simulink model "turbo_controller"  (R2025a)
settings: Solver=FixedStepAuto  StartTime=0.0  StopTime=inf  FixedStep=0.001  RelTol=1e-3
PostLoadFcn:
  | % 自动定位同目录CubeMX文件；不需要外部初始化脚本。
  | codertarget.data.setParameterValue('turbo_controller','STM32CubeMX.ProjectFile',fullfile(fileparts(get_param('turbo_controller','FileName')),'turbo_f407.ioc'));
InitFcn:
  | % 中文说明：按原控制器字段与类型创建三组接口总线；控制参数已内嵌。
  | tc_names=["EValve_Cycle" "EValve_Open" "Eblast_Cycle" "Eblast_Open" "Motor_Cycle" "Motor_Open" "EValve_Enable" "Eblast_Enable" "Motor_Enable" "SWO_Firework" "SWO_BleedAir" "EngineState" "Flag_ECUReset_Clear" "Flag_ECUReset_Save" "Flag_Reset_Enable" "Accelerator" "Nc_dem" "Nc"]; tc_types=["uint16" "uint16" "uint16" "uint16" "uint16" "uint16" "uint8" "uint8" "uint8" "uint8" "uint8" "uint8" "uint8" "uint8" "uint8" "single" "single" "single"];
  | for tc_k=1:numel(tc_names)
  |  tc_e(tc_k)=Simulink.BusElement; tc_e(tc_k).Name=char(tc_names(tc_k)); tc_e(tc_k).DataType=char(tc_types(tc_k));
  | end
  | EngineControl_Out=Simulink.Bus; EngineControl_Out.DataScope='Exported'; EngineControl_Out.Elements=tc_e;
  | clear tc_e tc_names tc_types tc_k
  | tc_names=["savedata1" "savedata2" "savedata3" "savedata4" "savedata5" "savedata6" "savedata7" "savedata8" "savedata9" "savedata10" "savedata11" "savedata12" "savedata13" "savedata14" "savedata15" "savedata16" "savedata17" "savedata18" "savedata19" "savedata20" "savedata21" "savedata22" "savedata23" "savedata24" "savedata25"]; tc_types=["single" "single" "single" "single" "single" "single" "single" "single" "single" "single" "single" "single" "single" "single" "single" "single" "single" "single" "single" "single" "single" "single" "single" "single" "single"];
  | for tc_k=1:numel(tc_names)
  |  tc_e(tc_k)=Simulink.BusElement; tc_e(tc_k).Name=char(tc_names(tc_k)); tc_e(tc_k).DataType=char(tc_types(tc_k));
  | end
  | SaveData_Out=Simulink.Bus; SaveData_Out.DataScope='Exported'; SaveData_Out.Elements=tc_e;
  | clear tc_e tc_names tc_types tc_k
  | tc_names=["senddata1" "senddata2" "senddata3" "senddata4" "senddata5" "senddata6" "senddata7" "senddata8" "senddata9" "senddata10" "senddata11" "senddata12" "senddata13" "senddata14" "senddata15" "senddata16" "senddata17" "senddata18" "senddata19" "senddata20" "senddata21" "senddata22" "senddata23" "senddata24" "senddata25" "senddata26" "senddata27" "senddata28" "senddata29"]; tc_types=["uint8" "uint8" "uint8" "uint8" "uint8" "uint8" "uint8" "uint8" "uint8" "uint8" "uint8" "uint8" "uint8" "uint8" "uint8" "uint8" "uint8" "uint8" "uint8" "uint8" "uint8" "uint8" "uint8" "uint8" "uint8" "uint8" "uint8" "uint8" "uint8"];
  | for tc_k=1:numel(tc_names)
  |  tc_e(tc_k)=Simulink.BusElement; tc_e(tc_k).Name=char(tc_names(tc_k)); tc_e(tc_k).DataType=char(tc_types(tc_k));
  | end
  | SendData_Out=Simulink.Bus; SendData_Out.DataScope='Exported'; SendData_Out.Elements=tc_e;
  | clear tc_e tc_names tc_types tc_k
  | 
  | % 以下为接口中文说明；只设置描述，不改变数值或数据类型。
  | EngineControl_Out.Description='执行控制输出（阀、电机、点火、状态及复位请求）';
  | tc_cn=["EValve_Cycle（主油阀周期计数（每计数2毫秒））" "EValve_Open（主油阀开通计数（每计数2毫秒））" "Eblast_Cycle（副油阀周期计数（每计数2毫秒））" "Eblast_Open（副油阀开通计数（每计数2毫秒））" "Motor_Cycle（起动电机周期计数）" "Motor_Open（起动电机开通计数）" "EValve_Enable（主油阀驱动使能）" "Eblast_Enable（副油阀驱动使能）" "Motor_Enable（起动电机使能）" "SWO_Firework（点火器使能（1开））" "SWO_BleedAir（引气阀使能（1开））" "EngineState（发动机状态）" "Flag_ECUReset_Clear（清除复位恢复状态请求）" "Flag_ECUReset_Save（保存复位恢复数据请求）" "Flag_Reset_Enable（处理器软件复位请求）" "Accelerator（油门／油泵给定控制量）" "Nc_dem（控制目标转速）" "Nc（发动机反馈转速（转每分））"];
  | tc_elements=EngineControl_Out.Elements;
  | for tc_k=1:numel(tc_cn)
  |  tc_elements(tc_k).Description=char(tc_cn(tc_k));
  | end
  | EngineControl_Out.Elements=tc_elements;
  | clear tc_cn tc_elements tc_k
  | SaveData_Out.Description='25项运行记录；字段含义按当前模型数据来源解释';
  | tc_cn=["savedata1（指令回显记录）" "savedata2（入口总温记录（℃））" "savedata3（电源电压记录）" "savedata4（排气温度记录（℃））" "savedata5（标定燃油压力记录）" "savedata6（副油阀占空比记录（％））" "savedata7（主油阀占空比记录（％））" "savedata8（温度修正转速记录）" "savedata9（开关输出及反馈位域）" "savedata10（物理转速记录）" "savedata11（油泵目标给定原始值）" "savedata12（起动电机占空比记录（％））" "savedata13（发动机状态码记录）" "savedata14（故障告警位域记录）" "savedata15（模型记录帧序号）" "savedata16（处理器温度记录（℃））" "savedata17（装订转速记录（沿用旧电源字段名））" "savedata18（导航高度记录）" "savedata19（飞行空速记录）" "savedata20（主阀旧记录位（恒零保留））" "savedata21（第21项保留记录（恒零））" "savedata22（保留记录项22）" "savedata23（保留记录项23）" "savedata24（保留记录项24）" "savedata25（保留记录项25）"];
  | tc_elements=SaveData_Out.Elements;
  | for tc_k=1:numel(tc_cn)
  |  tc_elements(tc_k).Description=char(tc_cn(tc_k));
  | end
  | SaveData_Out.Elements=tc_elements;
  | clear tc_cn tc_elements tc_k
  | SendData_Out.Description='29字段回传及外设命令接口；板端上位机帧只取第3至27字段';
  | tc_cn=["senddata1（回传发送允许标志（不直接上线路））" "senddata2（回传载荷长度25字节）" "senddata3（回传指令回显字节）" "senddata4（总温编码字节（℃＋80））" "senddata5（电源电压编码字节）" "senddata6（排温编码高字节）" "senddata7（排温编码低字节）" "senddata8（燃油压力编码高字节）" "senddata9（燃油压力编码低字节）" "senddata10（副油阀占空比字节（％））" "senddata11（主油阀占空比字节（％））" "senddata12（修正转速编码高字节）" "senddata13（修正转速编码低字节）" "senddata14（驱动及反馈状态位域）" "senddata15（物理转速编码高字节）" "senddata16（物理转速编码低字节）" "senddata17（油泵目标给定高字节（串口二使用））" "senddata18（油泵目标给定低字节（串口二使用））" "senddata19（起动电机占空比命令（串口一使用））" "senddata20（发动机状态码字节）" "senddata21（故障告警位域字节）" "senddata22（帧序号占位（板端另行填写））" "senddata23（处理器温度编码（℃＋50））" "senddata24（控制目标转速编码高字节）" "senddata25（控制目标转速编码低字节）" "senddata26（占位字节（板端改填实测泵速高字节））" "senddata27（占位字节（板端改填实测泵速低字节））" "senddata28（装订转速高字节（本板未发送））" "senddata29（装订转速低字节（本板未发送））"];
  | tc_elements=SendData_Out.Elements;
  | for tc_k=1:numel(tc_cn)
  |  tc_elements(tc_k).Description=char(tc_cn(tc_k));
  | end
  | SendData_Out.Elements=tc_elements;
  | clear tc_cn tc_elements tc_k
  | 
  | 
  | % FRAM模块化事务：接口类型和上电初始状态，随模型保存，无外部初始化文件。
  | clear FM_elements
  | FM_elements(1)=Simulink.BusElement;FM_elements(1).Name='phase';FM_elements(1).DataType='uint8';FM_elements(1).Dimensions=[1 1];FM_elements(1).Description='phase（当前事务阶段）';
  | FM_elements(2)=Simulink.BusElement;FM_elements(2).Name='a';FM_elements(2).DataType='uint8';FM_elements(2).Dimensions=[64 1];FM_elements(2).Description='a（启动时缓存的首区64字节）';
  | FM_elements(3)=Simulink.BusElement;FM_elements(3).Name='active';FM_elements(3).DataType='uint16';FM_elements(3).Dimensions=[1 1];FM_elements(3).Description='active（当前有效记录区地址）';
  | FM_elements(4)=Simulink.BusElement;FM_elements(4).Name='generation';FM_elements(4).DataType='uint32';FM_elements(4).Dimensions=[1 1];FM_elements(4).Description='generation（当前有效记录代号）';
  | FM_elements(5)=Simulink.BusElement;FM_elements(5).Name='record';FM_elements(5).DataType='uint8';FM_elements(5).Dimensions=[64 1];FM_elements(5).Description='record（本次冻结的待写记录）';
  | FM_elements(6)=Simulink.BusElement;FM_elements(6).Name='addr';FM_elements(6).DataType='uint16';FM_elements(6).Dimensions=[1 1];FM_elements(6).Description='addr（本次备用写入地址）';
  | FM_elements(7)=Simulink.BusElement;FM_elements(7).Name='lastSave';FM_elements(7).DataType='single';FM_elements(7).Dimensions=[1 1];FM_elements(7).Description='lastSave（上次开始保存的秒数）';
  | FM_elements(8)=Simulink.BusElement;FM_elements(8).Name='lastState';FM_elements(8).DataType='uint8';FM_elements(8).Dimensions=[1 1];FM_elements(8).Description='lastState（上次保存时的发动机状态）';
  | FM_elements(9)=Simulink.BusElement;FM_elements(9).Name='boot';FM_elements(9).DataType='boolean';FM_elements(9).Dimensions=[1 1];FM_elements(9).Description='boot（启动记录是否允许恢复）';
  | FM_elements(10)=Simulink.BusElement;FM_elements(10).Name='consumed';FM_elements(10).DataType='boolean';FM_elements(10).Dimensions=[1 1];FM_elements(10).Description='consumed（本次启动恢复通知是否已发送）';
  | FM_elements(11)=Simulink.BusElement;FM_elements(11).Name='payload';FM_elements(11).DataType='uint8';FM_elements(11).Dimensions=[20 1];FM_elements(11).Description='payload（当前20字节恢复内容）';
  | ... (+35 lines)
model workspace (MAT data in the model file):
  CRC16_Table_Reference = [0 4129 8258 12387 16516 20645 24774 28903 33032 37161 41290 45419 ... (256 elements, 256x1)]
  PE_Kaer = [0.15402 0.15402 0.12264 0.10076 0.09481 0.07601 0.07111 0.0569 0.05198 0.04926 0.05308 0.04325 ... (13 elements, 1x13)]
  PE_Nr = [21.2982 61.4260372 67.7475458 72.7394382 76.845934 80.6988798 83.8449282 86.6491912 88.9382406 89.178606 91.1938214 93.4068058 ... (13 elements, 1x13)]
  PE_Pump_Translate = 33.5999984741
  PE_RotaSpeed_Translate = 860
  PE_Taer = [0.4939154 0.4939154 0.40780982 0.34066978 0.31622756 0.30405716 0.34300244 0.26785022 0.37393554 0.23914836 0.44563948 0.31044662 ... (13 elements, 1x13)]
  PF_ACCFULLRANGE = 3360
  PF_Flag_ECUReset = 0
  PF_Flag_rx_suc = 1
  PF_Gear_Info = [40000; 45000; 50000; 55000; 57000; 59000; 60000; 61000; 61000; 61000; 61000; 61000]
  PF_K_TiaoJie = 1
  PF_Kpu = 10
  PF_MySet_Rxdata = [0 0 0 0 0 0 0 0 0 0 0 0 ... (50 elements, 50x1)]
  PF_MyUsart1_Rxdata = [0 0 0 0 0 0 0 0 0 0 0 0 ... (50 elements, 50x1)]
  PF_MyUsart2_Rxdata = [0 0 0 0 0 0 0 0 0 0 0 0 ... (50 elements, 50x1)]
  PF_Reset_Information = [0 0 0 0 0 0 0 0 0 0 0 0 ... (20 elements, 20x1)]
  PF_Sensor_X1_T4 = [0 4095]
  PF_Sensor_X2_T4 = [0 1.66666698456]
  PF_Sensor_X3_T4 = [0 504 999 1497 2010 2529 3051 3568 4076 4571 4959]
  PF_Sensor_X_P2 = [0.5 3]
  PF_Sensor_X_Poil = [0.5 3]
  PF_Sensor_X_T1t = [-50 300]
  PF_Sensor_X_Vpower = [0 3]
  PF_Sensor_X_Vpump = [0 3]
  PF_Sensor_Y1_T4 = [0 3]
  PF_Sensor_Y2_T4 = [0 5000]
  PF_Sensor_Y3_T4 = [0 100 200 300 400 500 600 700 800 900 980]
  PF_Sensor_Y_P2 = [0 1000]
  PF_Sensor_Y_Poil = [0 1000]
  PF_Sensor_Y_T1t = [-50 300]
  PF_Sensor_Y_Vpower = [0 33]
  PF_Sensor_Y_Vpump = [0 33]
  PG_CtrlMode_CloseLoop : mpt.Parameter (value not decoded)
  PG_CtrlMode_ManualAcc : mpt.Parameter (value not decoded)
  PG_CtrlMode_Origin : mpt.Parameter (value not decoded)
  PG_CtrlMode_Start : mpt.Parameter (value not decoded)
  PG_CtrlMode_Stop : mpt.Parameter (value not decoded)
  PG_ES_Clp : mpt.Parameter (value not decoded)
  PG_ES_EngStart : mpt.Parameter (value not decoded)
  PG_ES_Manual : mpt.Parameter (value not decoded)
  PG_ES_Origin : mpt.Parameter (value not decoded)
  PG_ES_Stop : mpt.Parameter (value not decoded)
  PG_Instr_BleedAirSet : mpt.Parameter (value not decoded)
  PG_Instr_CloseLoop : mpt.Parameter (value not decoded)
  PG_Instr_ECUReSet : mpt.Parameter (value not decoded)
  PG_Instr_EValveSet : mpt.Parameter (value not decoded)
  PG_Instr_EblastSet : mpt.Parameter (value not decoded)
  PG_Instr_Erase : mpt.Parameter (value not decoded)
  PG_Instr_FireWorkSet : mpt.Parameter (value not decoded)
  PG_Instr_ManualPlus : mpt.Parameter (value not decoded)
  PG_Instr_ManualrReduce : mpt.Parameter (value not decoded)
  PG_Instr_MotorSet : mpt.Parameter (value not decoded)
  PG_Instr_OilSet : mpt.Parameter (value not decoded)
  PG_Instr_SelfCheck : mpt.Parameter (value not decoded)
  PG_Instr_Start : mpt.Parameter (value not decoded)
  PG_Instr_Stop : mpt.Parameter (value not decoded)
  PG_Instr_StopZero : Simulink.Parameter (value not decoded)
  PG_Location_Air : Simulink.Parameter (value not decoded)
  PG_Location_Gnd : Simulink.Parameter (value not decoded)
  PG_ServoCtrlMode_CloseLoop : Simulink.Parameter (value not decoded)
  PG_ServoCtrlMode_CloseLoopMax : Simulink.Parameter (value not decoded)
  PG_ServoCtrlMode_CloseLoopMin : Simulink.Parameter (value not decoded)
  PG_ServoCtrlMode_ManualAcc : Simulink.Parameter (value not decoded)
  PG_ServoCtrlMode_ManualAccMax : Simulink.Parameter (value not decoded)
  PG_ServoCtrlMode_ManualAccMin : Simulink.Parameter (value not decoded)
  PG_SpeedDot_Permit : Simulink.Parameter (value not decoded)
  PL_EngineModel_Actuator = [0 10 100]
  PL_EngineModel_EngineStar_Press_P2 = [1013 1098.4 1099.144828 1099.931034 1103.613793 1162.662069 1143.793103 1131.006897 1123.186207 1117.6 1114 1111.806897 ... (127 elements, 1x127)]
  PL_EngineModel_EngineStar_RotaSpeed = [200 2000 9584 9660 10220 10240 10260 10288 10308 10368 10380 10408 ... (127 elements, 1x127)]
  PL_EngineModel_EngineStar_Temp_Exhaust = [128 129 129.1 130 131 131.1 132 133 134 134.1 135 135.1 ... (127 elements, 1x127)]
  PL_EngineModel_EngineStar_Time = [0.05 0.1 0.15 0.2 0.25 0.3 0.35 0.4 0.45 0.5 0.55 0.6 ... (127 elements, 1x127)]
  PL_EngineModel_IdleAbove_Nr = [0 21.2982 61.4260372 67.7475458 72.7394382 76.845934 80.6988798 83.8449282 86.6491912 88.9382406 89.178606 91.1938214 ... (14 elements, 1x14)]
  PL_EngineModel_IdleAbove_P2r = [0.986923266716 1.57907722675 1.81593881076 1.99358499877 2.23044658278 2.43770046879 2.65482358747 2.84233900814 3.03972366149 3.18776215149 3.25684678016 3.3950160375 ... (14 elements, 1x14)]
  PL_EngineModel_IdleAbove_Tempr = [0.0536001429337 1.07200285867 1.63301768805 1.63659103091 1.66875111667 1.72592460247 1.77595140254 1.86171163123 1.95461854565 2.03323208862 2.03323208862 2.13685903162 ... (14 elements, 1x14)]
  PL_EngineModel_IdleAbove_Ter = [0.42434128 0.42434128 0.42434128 0.30669408 0.23570008 0.22150128 0.1997974 0.23803274 0.16115638 0.24279948 0.13600422 0.31308354 ... (14 elements, 1x14)]
  PL_EngineModel_IdleAbove_Wfr = [0 10.142 23.8337 27.8905 31.9473 36.0041 40.0609 44.1177 48.1745 52.2313 52.7384 56.7952 ... (14 elements, 1x14)]
  PL_EngineModel_Press_P2 = [400 400 400 400 400 400 400 400 400 400]
  PL_EngineModel_Rotaspeed = [0 20000 96400]
  PL_EngineModel_Temp_Exhaust = [500 500 500 500 500 500 500 500 500 500]
  PL_Kaer = [0.1 0.1 0.1 0.1 0.1 0.1]
  PL_Nr = [50 60 70 80 90 100]
  PL_Taer = [0.1 0.1 0.1 0.1 0.1 0.1]
  Sig : Simulink.Signal (value not decoded)
  Ts_ms : Simulink.Parameter (value not decoded)
  false : Simulink.Parameter (value not decoded)
  true : Simulink.Parameter (value not decoded)
symbols that are objects in the model workspace (value not decoded): PG_CtrlMode_CloseLoop, PG_CtrlMode_ManualAcc, PG_CtrlMode_Origin, PG_CtrlMode_Start, PG_CtrlMode_Stop, PG_ES_Clp, PG_ES_EngStart, PG_ES_Manual, PG_ES_Origin, PG_ES_Stop, PG_Instr_BleedAirSet, PG_Instr_CloseLoop, PG_Instr_EblastSet, PG_Instr_ECUReSet, PG_Instr_Erase, PG_Instr_EValveSet, PG_Instr_FireWorkSet, PG_Instr_ManualPlus, PG_Instr_ManualrReduce, PG_Instr_MotorSet, PG_Instr_OilSet, PG_Instr_SelfCheck, PG_Instr_Start, PG_Instr_Stop, PG_Instr_StopZero, PG_ServoCtrlMode_CloseLoop, PG_ServoCtrlMode_CloseLoopMax, PG_ServoCtrlMode_CloseLoopMin, PG_ServoCtrlMode_ManualAcc, PG_ServoCtrlMode_ManualAccMax, PG_ServoCtrlMode_ManualAccMin, Ts_ms
libraries: simulink x97, stm32blockslib x10, stm32f4xxblockslib x8
(part 16 of 26)

== system turbo_controller/COMMRead_ISM/ECUReset_Information_Read/ECUReset_Acclerator_Cal ==
  note: 把保存的两个字节还原成油泵给定
      |
      | 按高字节在前合成：泵给定=高字节×256+低字节。例如高字节11、低字节184，恢复得到3000。
      |
      | 这里只恢复无符号控制编码，不换算成燃油流量，不根据电压补偿，也不验证整条FRAM记录。记录校验
      | 、恢复是否允许和最终是否采用该值在事务层及父级完成。输入字段位置按恢复信息协议排列，不能随
      | 意调换高低字节。
  S_ECUReset_Information : Inport
      settings: AttributesFormatString=S_ECUReset_Information（铁电存储器中的复位恢复记录）
  ECUReset_Information_Acclerator1 : Selector  IndexMode=Zero-based  InputPortWidth=20  IndexOptions=Index vector (dialog)  Indices=[6]  OutputSizes=1
      settings: AttributesFormatString=ECUReset_Information_Acclerator1（控制器复位信息油门1）
  ECUReset_Information_Acclerator2 : Selector  IndexMode=Zero-based  InputPortWidth=20  IndexOptions=Index vector (dialog)  Indices=[7]  OutputSizes=1
      settings: AttributesFormatString=ECUReset_Information_Acclerator2（控制器复位信息油门2）
  Product20 : Product  Inputs=**
      settings: AttributesFormatString=Product20（乘法20）
  Sum of Elements3 : Sum
      settings: AttributesFormatString=Sum of Elements3（加法求和的元素3）
  dth = T0-288.24 : Constant  Value=256  OutDataTypeStr=single  SampleTime=-1
      settings: AttributesFormatString=dth = T0-288.24（固定常量256（旧名称不参与计算））
  S_ECUReset_Acclerator : Outport
      settings: AttributesFormatString=S_ECUReset_Acclerator（电子控制器复位油门）
  wires:
  Sum of Elements3/1 -> S_ECUReset_Acclerator/1
  ECUReset_Information_Acclerator1/1 -> Product20/1
  dth = T0-288.24/1 -> Product20/2
  Product20/1 -> Sum of Elements3/1
  ECUReset_Information_Acclerator2/1 -> Sum of Elements3/2
  S_ECUReset_Information/1 -> ECUReset_Information_Acclerator2/1, ECUReset_Information_Acclerator1/1

== system turbo_controller/COMMRead_ISM/ECUReset_Information_Read/Flag_ECUReset_Manage ==
  note: 还原保存的目标转速，并判定可否采用
      |
      | 从恢复信息中取出三个字节，高字节在前合成：
      | 目标rpm=高字节×65536+中字节×256+低字节。
      | 例如0、195、80合成50000。
      |
      | 目标在30000～89000之间才满足本模块的数值范围要求，再与外部恢复有效标志组合，形成恢复使用许
      | 可。范围合法仅说明数值像一个允许的目标，不能代替FRAM记录校验；外部标志为假时仍不采用。
      |
      | 目标输出继续送SpeedLoad_Analyse，最终还取决于当前模式和恢复选择。当前上层使能固定false，因
      | 此本模块的解码结果不会自行激活闭环。
  S_ECUReset_Information : Inport
      settings: AttributesFormatString=S_ECUReset_Information（铁电存储器中的复位恢复记录）
  S_Flag_ECUReset : Inport  Port=2
      settings: AttributesFormatString=S_Flag_ECUReset（复位恢复标志）
  ECUReset_Information_NcDem1 : Selector  IndexMode=Zero-based  InputPortWidth=20  IndexOptions=Index vector (dialog)  Indices=[10]  OutputSizes=1
      settings: AttributesFormatString=ECUReset_Information_NcDem1（控制器复位信息目标转速1）
  ECUReset_Information__NcDem2 : Selector  IndexMode=Zero-based  InputPortWidth=20  IndexOptions=Index vector (dialog)  Indices=[11]  OutputSizes=1
      settings: AttributesFormatString=ECUReset_Information__NcDem2（控制器复位信息目标转速2）
  ECUReset_Information__NcDem3 : Selector  IndexMode=Zero-based  InputPortWidth=20  IndexOptions=Index vector (dialog)  Indices=[12]  OutputSizes=1
      settings: AttributesFormatString=ECUReset_Information__NcDem3（控制器复位信息目标转速3）
  Logical Operator2 : Logic  AllPortsSameDT=off  OutDataTypeStr=boolean
      settings: AttributesFormatString=Logical Operator2（逻辑运算2）
  Logical Operator_ReSet : Logic  AllPortsSameDT=off  OutDataTypeStr=boolean
      settings: AttributesFormatString=Logical Operator_ReSet（逻辑运算复位）
  Product1 : Product  Inputs=**
      settings: AttributesFormatString=Product1（乘法1）
  Product2 : Product  Inputs=**
      settings: AttributesFormatString=Product2（乘法2）
  Relational Operator1 : RelationalOperator  OutDataTypeStr=boolean  InputSameDT=off
      settings: AttributesFormatString=Relational Operator1（关系比较运算1）
  Relational Operator6 : RelationalOperator  Operator=<=  OutDataTypeStr=boolean  InputSameDT=off
      settings: AttributesFormatString=Relational Operator6（关系比较运算6）
  Sum of Elements1 : Sum  Inputs=+++
      settings: AttributesFormatString=Sum of Elements1（加法求和的元素1）
  ZhuangDingShangXian_uint32 : Constant  Value=89000  OutDataTypeStr=uint32
      settings: AttributesFormatString=ZhuangDingShangXian_uint32（装订上限三十二位无符号整数）
  ZhuangDingXiaXian_uint32 : Constant  Value=30000  OutDataTypeStr=uint32
      settings: AttributesFormatString=ZhuangDingXiaXian_uint32（装订下限三十二位无符号整数）
  dth = T0-288.1 : Constant  Value=256  OutDataTypeStr=single  SampleTime=-1
      settings: AttributesFormatString=dth = T0-288.1（固定常量256（旧名称不参与计算））
  dth = T0-288.2 : Constant  Value=65536  OutDataTypeStr=single  SampleTime=-1
      settings: AttributesFormatString=dth = T0-288.2（固定常量65536（旧名称不参与计算））
  S_Flag_ECUReset_Process : Outport
      settings: AttributesFormatString=S_Flag_ECUReset_Process（标志控制器复位处理）
  S_ECUReset_NcDem : Outport  Port=2
      settings: AttributesFormatString=S_ECUReset_NcDem（电子控制器复位目标转速）
  wires:
  Logical Operator2/1 -> S_Flag_ECUReset_Process/1
  S_ECUReset_Information/1 -> ECUReset_Information_NcDem1/1, ECUReset_Information__NcDem3/1, ECUReset_Information__NcDem2/1
  Relational Operator6/1 -> Logical Operator_ReSet/2
  Relational Operator1/1 -> Logical Operator_ReSet/1
  ZhuangDingShangXian_uint32/1 -> Relational Operator6/2
  ZhuangDingXiaXian_uint32/1 -> Relational Operator1/2
  dth = T0-288.1/1 -> Product1/2
  ECUReset_Information__NcDem2/1 -> Product1/1
  ECUReset_Information__NcDem3/1 -> Sum of Elements1/3
  Product1/1 -> Sum of Elements1/2
  Product2/1 -> Sum of Elements1/1
  ECUReset_Information_NcDem1/1 -> Product2/1
  dth = T0-288.2/1 -> Product2/2
  Sum of Elements1/1 -> S_ECUReset_NcDem/1, Relational Operator6/1, Relational Operator1/1
  Logical Operator_ReSet/1 -> Logical Operator2/1
  S_Flag_ECUReset/1 -> Logical Operator2/2

== system turbo_controller/COMMRead_ISM/ISM/AnalogFilter_Nc ==
  note: 检查转速可信度，并形成控制转速及相对转速
      |
      | 先按模式设置转速下限：闭环时采用10000，其他模式采用0；上限70000。GeneralFilter同时检查相邻
      | 两拍变化，突变量门限1200、恢复门限800、恢复确认参数100 ms。
      |
      | 异常样本可能被上一有效值替代，然后进行一阶低通，得到Nc_Filter。范围故障与变化故障分别输出
      | ，供FPM决定暂时保持控制还是采用故障备份曲线。
      |
      | 相对转速以61000 rpm为100%：百分比=当前转速×100/61000。另有按温度sqrt(288.15/T1t_calc)修正
      | 的转速及百分比。温度必须为K；当前此输入由上层接288.15 K，修正系数为1。不要与独立的ADC总温
      | 修正记录通道混淆。
  T1t_calc : Inport
      settings: AttributesFormatString=T1t_calc（入口总温计算）
  S_Nc : Inport  Port=2
      settings: AttributesFormatString=S_Nc（发动机反馈转速（转每分））
  S_EngineState : Inport  Port=3
      settings: AttributesFormatString=S_EngineState（发动机状态）
  Constant1 : Constant  Value=0  OutDataTypeStr=single  SampleTime=-1
      settings: AttributesFormatString=Constant1（常量1）
  Constant2 : Constant  Value=70000  OutDataTypeStr=single  SampleTime=-1
      settings: AttributesFormatString=Constant2（常量2）
  Constant3 : Constant  Value=10000  OutDataTypeStr=single  SampleTime=-1
      settings: AttributesFormatString=Constant3（常量3）
  Constant4 : Constant  Value=1200  OutDataTypeStr=single  SampleTime=-1
      settings: AttributesFormatString=Constant4（常量4）
  Constant5 : Constant  Value=800  OutDataTypeStr=single  SampleTime=-1
      settings: AttributesFormatString=Constant5（常量5）
  Constant6 : Constant  Value=100  OutDataTypeStr=single  SampleTime=-1
      settings: AttributesFormatString=Constant6（常量6）
  GeneralFilter : Subsystem  Description=|  RequirementInfo={} %GIDa_36ea9eb8_e302_4863_9c8a_4518a6f49dc1
      | 先拒绝明显不可信的转速，再平滑有效值
      | 
      | Xlim_Xdot_Judge比较当前原始输入、前一拍原始输入和前一拍有效输出。超出允许上下限或突变不满足接受条件时，输出沿用上次有效值，并分别标记幅值故障、变化故障。
      | 
      | 恢复时不仅要求变化回到较小门限，还要达到连续确认次数。次数由恢复时间/Ts_ms计算，避免一拍恢复就马上解除故障。
      | 
      | 通过检查的值再进入一阶低通，延迟同时保存本拍原始值和有效值，供下一拍比较。因此“原始上一拍”与“上一有效输出”是两条不同的记忆，不能混为一个变量。
      settings: AttributesFormatString=GeneralFilter（通用滤波）
  N1r_idle1 : Constant  Value=PG_ES_Clp  OutDataTypeStr=uint8  SampleTime=-1
      settings: AttributesFormatString=N1r_idle1（一级转速归一化值慢车1）
  Product1 : Product  Inputs=**/
      settings: AttributesFormatString=Product1（乘法1）
  Product2 : Product  Inputs=*/
      settings: AttributesFormatString=Product2（乘法2）
  Product3 : Product  Inputs=**
      settings: AttributesFormatString=Product3（乘法3）
  Product4 : Product  Inputs=**
      settings: AttributesFormatString=Product4（乘法4）
  Relational Operator4 : RelationalOperator  Operator===  OutDataTypeStr=boolean  InputSameDT=off
      settings: AttributesFormatString=Relational Operator4（关系比较运算4）
  Sqrt : Sqrt
      settings: AttributesFormatString=Sqrt（平方根）
  Switch : Switch  Criteria=u2 ~= 0  SaturateOnIntegerOverflow=off  InputSameDT=off
      settings: AttributesFormatString=Switch（开关选择）
  constant1 : Constant  Value=single(288.15)  OutDataTypeStr=single  SampleTime=-1
      settings: AttributesFormatString=constant1（常量1）
  constant2 : Constant  Value=100  OutDataTypeStr=single  SampleTime=-1
      settings: AttributesFormatString=constant2（常量2）
  constant3 : Constant  Value=61000  OutDataTypeStr=single  SampleTime=-1
      settings: AttributesFormatString=constant3（常量3）
  Nc_Flag_Locking : Outport
      settings: AttributesFormatString=Nc_Flag_Locking（转速标志锁存）
  Ncdot_Flag_Locking : Outport  Port=2
      settings: AttributesFormatString=Ncdot_Flag_Locking（控制器转速变化量标志锁存）
  Nc_Filter : Outport  Port=3
      settings: AttributesFormatString=Nc_Filter（滤波后的转速）
  Nc_Percent : Outport  Port=4
      settings: AttributesFormatString=Nc_Percent（转速百分比）
  Ncr : Outport  Port=5
      settings: AttributesFormatString=Ncr（归一化控制器转速）
  Ncr_Percent : Outport  Port=6
      settings: AttributesFormatString=Ncr_Percent（归一化控制器转速百分比）
  wires:
  GeneralFilter/3(S_Xout) -> Product3/1, Product1/1, Nc_Filter/1  "Nc（反馈转速）"
  Constant4/1 -> GeneralFilter/4(Xdot_lim)
  GeneralFilter/1(S_X_Flag_Locking) -> Nc_Flag_Locking/1  "X_Flag_Locking（输入信号锁定标志）"
  Constant2/1 -> GeneralFilter/2(X_ulim)
  S_Nc/1 -> GeneralFilter/1(Xin)
  Constant6/1 -> GeneralFilter/6(Xdot_CancelTime)
  GeneralFilter/2(S_Xdot_Flag_Locking) -> Ncdot_Flag_Locking/1  "Xdot_Flag_Locking（输入变化率锁定标志）"
  Switch/1 -> GeneralFilter/3(X_llim)
  Constant5/1 -> GeneralFilter/5(Xdot_CancelLim)
  Product1/1 -> Product4/1, Nc_Percent/1  "Nc_Percent（转速百分比）"
  constant2/1 -> Product1/2
  constant3/1 -> Product1/3
  constant1/1 -> Product2/1
  T1t_calc/1 -> Product2/2
  Product2/1 -> Sqrt/1
  Sqrt/1 -> Product3/2, Product4/2
  Product4/1 -> Ncr_Percent/1  "Ncr_Percent（归一化控制器转速百分比）"
  Product3/1 -> Ncr/1  "Ncr（归一化控制器转速）"
  N1r_idle1/1 -> Relational Operator4/2
  S_EngineState/1 -> Relational Operator4/1
  Constant1/1 -> Switch/3
  Constant3/1 -> Switch/1
  Relational Operator4/1 -> Switch/2

== system turbo_controller/COMMRead_ISM/ISM/AnalogFilter_Poil ==
  note: 对标定后的油压做一阶低通，减小采样抖动
      |
      | 每次把本拍输入与上次滤波结果按比例相加：
      | 本拍输出=α×本拍输入+β×上次输出；
      | α=Ts/(T+Ts)，β=T/(T+Ts)。
      |
      | 当前T=0.067 s，Ts=Ts_ms/1000=0.02 s，因此α约0.229885、β约0.770115。新输入约占23%，旧结果
      | 约占77%。例如上次输出100、本次输入200，本次滤波结果约123，随后逐步靠近200。
      |
      | 它抑制快速波动，也会让真实变化稍有滞后；不负责把ADC计数变成物理量，也不单凭滤波判定传感器
      | 故障。输出送POil_Filter，供起动阶段比较压力建立情况并用于记录。
  In1 : Inport
      settings: AttributesFormatString=In1（输入1）
  Constant7 : Constant  Value=Ts_ms  OutDataTypeStr=single  SampleTime=-1
      settings: AttributesFormatString=Constant7（常量7）
  Constant8 : Constant  Value=1000  OutDataTypeStr=single  SampleTime=-1
      settings: AttributesFormatString=Constant8（常量8）
  Constant9 : Constant  Value=single(0.067)  OutDataTypeStr=single  SampleTime=-1
      settings: AttributesFormatString=Constant9（常量9）
  Divide : Product  Inputs=*/
      settings: AttributesFormatString=Divide（除法）
  Integer Delay1 : Delay  DelayLength=1  InitialCondition=0
      settings: AttributesFormatString=Integer Delay1（整数延迟1）
  Product2 : Product  RndMeth=Zero
      settings: AttributesFormatString=Product2（乘法2）
  Product3 : Product  RndMeth=Zero
      settings: AttributesFormatString=Product3（乘法3）
  Subsystem1 : Subsystem  Description=|
      | 计算低通滤波中新样本的权重
      | 
      | 输入T为滤波时间常数（s），T_Sampling为采样周期（s）。输出α=T_Sampling/(T+T_Sampling)，供父级乘以本拍的新输入。
      | 
      | 当前T=0.067、采样周期0.02，α=0.02/0.087≈0.229885。也就是每拍只采用约23%的新值，另外约77%由历史结果补足。时间常数越大，新值权重越小，结果越平稳但响应越慢。
      | 
      | 本模块只算一个无量纲系数，不含延迟，也不直接输出温度、压力或转速。两项时间输入必须使用同一单位。
      settings: AttributesFormatString=Subsystem1（子系统1）
      mask Display: disp('T_S\n---------------\nT_S + T')
  Subsystem2 : Subsystem  Description=|
      | 计算低通滤波中历史结果的权重
      | 
      | 输入T为时间常数，T_Sampling为采样周期，两者都用s。输出β=T/(T+T_Sampling)，供父级乘以上一次滤波结果。
      | 
      | 当前T=0.067、采样周期0.02，β≈0.770115；与另一支路新样本权重α≈0.229885相加为1。这样常值输入最终会稳定在原值，不会因为反复相加而不断放大。
      | 
      | 本模块只计算系数，历史结果由父级延迟块保存。若把20 ms误传成20 s，权重和滤波速度都会完全改变，因此父级先将Ts_ms除以1000。
      settings: AttributesFormatString=Subsystem2（子系统2）
      mask Display: disp('T\n---------------\nT_S + T')
  Sum3 : Sum  Inputs=|++
      settings: AttributesFormatString=Sum3（加法求和3）
  POil_Filter : Outport
      settings: AttributesFormatString=POil_Filter（油压滤波）
  wires:
  Sum3/1 -> POil_Filter/1, Integer Delay1/1
  In1/1 -> Product2/1
  Constant9/1 -> Subsystem2/1(T), Subsystem1/1(T)  "T（滤波时间常数）"
  Subsystem1/1(Out) -> Product2/2
  Product2/1 -> Sum3/1
  Product3/1 -> Sum3/2
  Subsystem2/1(Out) -> Product3/2
  Integer Delay1/1 -> Product3/1
  Constant7/1 -> Divide/1
  Divide/1 -> Subsystem2/2(T_Sampling), Subsystem1/2(T_Sampling)  "T_S（采样周期）"
  Constant8/1 -> Divide/2

== system turbo_controller/COMMRead_ISM/ISM/AnalogFilter_T4 ==
  note: 对标定后的排温做一阶低通，减小采样抖动
      |
      | 每次把本拍输入与上次滤波结果按比例相加：
      | 本拍输出=α×本拍输入+β×上次输出；
      | α=Ts/(T+Ts)，β=T/(T+Ts)。
      |
      | 当前T=0.067 s，Ts=Ts_ms/1000=0.02 s，因此α约0.229885、β约0.770115。新输入约占23%，旧结果
      | 约占77%。例如上次输出100、本次输入200，本次滤波结果约123，随后逐步靠近200。
      |
      | 它抑制快速波动，也会让真实变化稍有滞后；不负责把ADC计数变成物理量，也不单凭滤波判定传感器
      | 故障。输出送T4_Filter，供起动、告警与记录。
  In1 : Inport
      settings: AttributesFormatString=In1（输入1）
  Constant7 : Constant  Value=Ts_ms  OutDataTypeStr=single  SampleTime=-1
      settings: AttributesFormatString=Constant7（常量7）
  Constant8 : Constant  Value=1000  OutDataTypeStr=single  SampleTime=-1
      settings: AttributesFormatString=Constant8（常量8）
  Constant9 : Constant  Value=single(0.067)  OutDataTypeStr=single  SampleTime=-1
      settings: AttributesFormatString=Constant9（常量9）
  Divide : Product  Inputs=*/
      settings: AttributesFormatString=Divide（除法）
  Integer Delay1 : Delay  DelayLength=1  InitialCondition=0
      settings: AttributesFormatString=Integer Delay1（整数延迟1）
  Product2 : Product  RndMeth=Zero
      settings: AttributesFormatString=Product2（乘法2）
  Product3 : Product  RndMeth=Zero
      settings: AttributesFormatString=Product3（乘法3）
  Subsystem1 : Subsystem  Description=|
      | 计算低通滤波中新样本的权重
      | 
      | 输入T为滤波时间常数（s），T_Sampling为采样周期（s）。输出α=T_Sampling/(T+T_Sampling)，供父级乘以本拍的新输入。
      | 
      | 当前T=0.067、采样周期0.02，α=0.02/0.087≈0.229885。也就是每拍只采用约23%的新值，另外约77%由历史结果补足。时间常数越大，新值权重越小，结果越平稳但响应越慢。
      | 
      | 本模块只算一个无量纲系数，不含延迟，也不直接输出温度、压力或转速。两项时间输入必须使用同一单位。
      settings: AttributesFormatString=Subsystem1（子系统1）
      mask Display: disp('T_S\n---------------\nT_S + T')
  Subsystem2 : Subsystem  Description=|
      | 计算低通滤波中历史结果的权重
      | 
      | 输入T为时间常数，T_Sampling为采样周期，两者都用s。输出β=T/(T+T_Sampling)，供父级乘以上一次滤波结果。
      | 
      | 当前T=0.067、采样周期0.02，β≈0.770115；与另一支路新样本权重α≈0.229885相加为1。这样常值输入最终会稳定在原值，不会因为反复相加而不断放大。
      | 
      | 本模块只计算系数，历史结果由父级延迟块保存。若把20 ms误传成20 s，权重和滤波速度都会完全改变，因此父级先将Ts_ms除以1000。
      settings: AttributesFormatString=Subsystem2（子系统2）
      mask Display: disp('T\n---------------\nT_S + T')
  Sum3 : Sum  Inputs=|++
      settings: AttributesFormatString=Sum3（加法求和3）
  T4_Filter : Outport
      settings: AttributesFormatString=T4_Filter（滤波排温）
  wires:
  Sum3/1 -> T4_Filter/1, Integer Delay1/1
  In1/1 -> Product2/1
  Constant9/1 -> Subsystem2/1(T), Subsystem1/1(T)  "T（滤波时间常数）"
  Subsystem1/1(Out) -> Product2/2
  Product2/1 -> Sum3/1
  Product3/1 -> Sum3/2
  Subsystem2/1(Out) -> Product3/2
  Integer Delay1/1 -> Product3/1
  Constant7/1 -> Divide/1
  Divide/1 -> Subsystem2/2(T_Sampling), Subsystem1/2(T_Sampling)  "T_S（采样周期）"
  Constant8/1 -> Divide/2

== system turbo_controller/COMMRead_ISM/ISM/Calibrating_Poil ==
  note: 油压计数怎样换成压力
      |
      | 输入来自BoardInput的ADC第8项，仍是single类型的ADC计数。本模块依次经过两张线性查表，输出压
      | 力工程量，随后交给AnalogFilter_Poil平滑。
      |
      | 第一张Bit2V表把0～4095计数映射为0～3.3 V：
      | 传感器电压 = ADC计数 × 3.3 / 4095。
      | 第二张POil_X_Y表采用0.5 V对应0、3.0 V对应1000：
      | 压力 = (传感器电压 - 0.5) / 2.5 × 1000。
      |
      | 例如电压为1.75 V时，恰好在0.5和3.0 V中点，得到压力500。两张表超出断点时都采用端点值，所以
      | 最终量程为0～1000，而不是继续向表外延伸。
      |
      | 这里能从参数确定量程，压力单位应与实际传感器和工程约定对应。本模块没有做滤波，也没有生成油
      | 压故障标志；这些不能从“标定”二字推断出来。下一级滤波后的POil_Filter用于原位、普通起动、
      | 记录和回传。
  In1 : Inport
      settings: AttributesFormatString=In1（油压采样码入口（板端单位待核））
  Bit2V : Lookup_n-D  NumberOfTableDimensions=1  BreakpointsForDimension1=[0.0 4095.0]  BreakpointsForDimension2=1  BreakpointsForDimension3=1  Table=single([0.0 3.3])  ExtrapMethod=Clip  UseLastTableValue=on  InternalRulePriority=Speed  RndMeth=Simplest
      settings: AttributesFormatString=Bit2V（ADC采样码换算电压）
  POil_X_Y : Lookup_n-D  NumberOfTableDimensions=1  BreakpointsForDimension1=PF_Sensor_X_Poil  BreakpointsForDimension2=1  BreakpointsForDimension3=1  Table=PF_Sensor_Y_Poil  ExtrapMethod=Clip  UseLastTableValue=on  InternalRulePriority=Speed  RndMeth=Simplest
      settings: AttributesFormatString=POil_X_Y（油压自变量或输入量因变量或输出量）
  out : Outport
      settings: AttributesFormatString=out（标定燃油压力输出）
  wires:
  POil_X_Y/1 -> out/1
  In1/1 -> Bit2V/1
  Bit2V/1 -> POil_X_Y/1

== system turbo_controller/COMMRead_ISM/ISM/Calibrating_T0 ==
  note: 把总温编码还原成摄氏温度
      |
      | 输入来自BoardInput/TotalTemperature。那一路已用两路ADC反算电阻并计算温度，但为了沿用接口格
      | 式，输出时额外加了80。本模块先减掉这个偏置：
      | 摄氏总温 = 输入编码 - 80。
      |
      | 随后Range把结果限制在-70～175 ℃。例如输入105，减80后得到25 ℃；输入300，原结果220 ℃超过
      | 上限，最后输出175 ℃。限幅只是约束数值范围，不会单独输出断线或超温故障。
      |
      | 处理后的Sensor.T0一路给SaveData和SendData记录回传，另一路给HuanSuanN，与原位滤波转速计算温
      | 度修正转速。本模块没有独立低通滤波。
      | 注意：上游无效电压差可能被替代为R=9999，最终也会走到175 ℃上限，因此175 ℃可能是限幅/替代
      | 结果。
  In1 : Inport
      settings: AttributesFormatString=In1（总温加80编码入口）
  Constant5 : Constant  Value=175  OutDataTypeStr=single
      settings: AttributesFormatString=Constant5（常量5）
  Constant6 : Constant  Value=-70  OutDataTypeStr=single
      settings: AttributesFormatString=Constant6（常量6）
  Range : Stateflow chart  Description=|  TreatAsAtomicUnit=on
      | 本实例限制T0在-70～175 ℃。总温编码减80后若为9999等大值，最终显示175；这属于上限截断，不代表真实温度就是175 ℃，本处未另行产生总温故障标志。
      | 
      | 把一个数限制在允许范围内
      | 
      | 输入包括待处理值、允许下限和允许上限。先比较是否越过上限，越过就输出上限；未超过上限时再检查下限，小于下限就输出下限；落在范围内则原样通过。恰好等于边界的值也保留。
      | 
      | 计算式：输出 = min(max(输入，下限)，上限)。
      | 例如下限为0、上限为100时，输入120输出100，输入-5输出0，输入60输出60。这里不做平均、不计算变化速度，也不记住上一拍；它只防止当前数值越界。具体边界由父子系统连入，不能把此处的输出一律理解为百分比。
      settings: AttributesFormatString=Range（限幅或范围）
  Sum of Elements : Sum  Inputs=+-
      settings: AttributesFormatString=Sum of Elements（加法求和的元素）
  V25 : Constant  Value=80  OutDataTypeStr=single
      settings: AttributesFormatString=V25（总温编码偏移80℃）
  out : Outport
      settings: AttributesFormatString=out（总温解码输出（℃））
  wires:
  In1/1 -> Sum of Elements/1
  V25/1 -> Sum of Elements/2
  Sum of Elements/1 -> Range/1(In)
  Constant6/1 -> Range/3(Min)
  Constant5/1 -> Range/2(Max)
  Range/1(Out) -> out/1

== system turbo_controller/COMMRead_ISM/ISM/Calibrating_T4 ==
  note: 排温计数怎样经过三级标定
      |
      | 输入来自ADC第4项，BoardInput仅完成single转换。当前计数依次经过三张表，而不是直接乘一个温度
      | 系数。
      |
      | 第一张T4_X1_Y1把0～4095计数映射到0～3 V，等价于V=计数×3/4095。
      | 第二张T4_X2_Y2把0～约1.666667 V映射到0～5000的传感器标定中间量；这仍不是摄氏温度。
      | 第三张T4_X3_Y3根据非线性标定表，把中间量换成排温。例如中间量504对应100 ℃、999对应200 ℃、
      | 2529对应500 ℃、4959对应980 ℃。504是第三级表的输入，不是原ADC计数。
      |
      | 每张表在相邻断点间线性插值：输出=左端输出+(右端输出-左端输出)×当前位置比例。若输入超出表范
      | 围，采用该表端点值。这样分别表达电路比例和传感器非线性。
      |
      | 输出排温分两路：一路送AnalogFilter_T4作0.067 s一阶滤波，供起动、停车、冷吹和850 ℃告警；另
      | 一路在滤波前送Subsystem2作930 ℃超限判断。这里没有直接驱动阀门，也没有直接发停车命令。
  In1 : Inport
      settings: AttributesFormatString=In1（排温ADC采样码入口）
  T4_X1_Y1 : Lookup_n-D  NumberOfTableDimensions=1  BreakpointsForDimension1=PF_Sensor_X1_T4  BreakpointsForDimension2=1  BreakpointsForDimension3=1  Table=PF_Sensor_Y1_T4  ExtrapMethod=Clip  UseLastTableValue=on  InternalRulePriority=Speed  RndMeth=Simplest
      settings: AttributesFormatString=T4_X1_Y1（排温采样码转电压）
  T4_X2_Y2 : Lookup_n-D  NumberOfTableDimensions=1  BreakpointsForDimension1=PF_Sensor_X2_T4  BreakpointsForDimension2=1  BreakpointsForDimension3=1  Table=PF_Sensor_Y2_T4  ExtrapMethod=Clip  UseLastTableValue=on  InternalRulePriority=Speed  RndMeth=Simplest
      settings: AttributesFormatString=T4_X2_Y2（排温电压转热电势）
  T4_X3_Y3 : Lookup_n-D  NumberOfTableDimensions=1  BreakpointsForDimension1=PF_Sensor_X3_T4  BreakpointsForDimension2=1  BreakpointsForDimension3=1  Table=PF_Sensor_Y3_T4  ExtrapMethod=Clip  UseLastTableValue=on  InternalRulePriority=Speed  RndMeth=Simplest
      settings: AttributesFormatString=T4_X3_Y3（热电势查表转排温）
  out : Outport
      settings: AttributesFormatString=out（标定排温输出（℃））
  wires:
  T4_X3_Y3/1 -> out/1
  In1/1 -> T4_X1_Y1/1
  T4_X2_Y2/1 -> T4_X3_Y3/1
  T4_X1_Y1/1 -> T4_X2_Y2/1

== system turbo_controller/COMMRead_ISM/ISM/Calibrating_Tecu ==
  note: 芯片内部温度计数怎样换成摄氏温度
      |
      | 输入是ADC数组第3项，对应STM32内部温度传感器。它不是排气温度，也不是环境总温。
      |
      | 先用Bit2V表把0～4095计数映射到0～3.0 V，得到传感器电压V。随后按当前模型的参考点和斜率计算
      | ：
      | Tecu = (V - 0.76) × 400 + 25，单位℃。
      |
      | 0.76 V对应25 ℃；电压比参考值增加0.01 V时，按本公式温度增加4 ℃。这里的400是当前采用的摄氏
      | 度/伏特比例，实际标定是否适合硬件要以传感器参数为依据。
      |
      | 输出组成Sensor.Tecu，主要交给SaveData记录和SendData回传。当前没有查到独立的控制器过温停车
      | 分支，也没有在这里低通滤波。SendData会加50、限制到0～255，再变成字节；例如25 ℃回传编码约
      | 为75。
  In1 : Inport
      settings: AttributesFormatString=In1（处理器温度ADC采样码入口）
  " Avg_Slope" : Constant  Value=400  OutDataTypeStr=single
      settings: AttributesFormatString=Avg_Slope（平均斜率）
  " Avg_Slope1" : Constant  Value=25  OutDataTypeStr=single
      settings: AttributesFormatString=Avg_Slope1（平均斜率1）
  Bit2V : Lookup_n-D  NumberOfTableDimensions=1  BreakpointsForDimension1=[0.0 4095.0]  BreakpointsForDimension2=1  BreakpointsForDimension3=1  Table=[0.0 3.0]  ExtrapMethod=Clip  UseLastTableValue=on  InternalRulePriority=Speed  RndMeth=Simplest
      settings: AttributesFormatString=Bit2V（ADC采样码换算电压）
  Divide : Product  Inputs=**
      settings: AttributesFormatString=Divide（除法）
  Sum of Elements : Sum  Inputs=+-
      settings: AttributesFormatString=Sum of Elements（加法求和的元素）
  Sum of Elements1 : Sum
      settings: AttributesFormatString=Sum of Elements1（加法求和的元素1）
  V25 : Constant  Value=single(0.76)  OutDataTypeStr=single
      settings: AttributesFormatString=V25（25℃参考电压0.76伏）
  out : Outport
      settings: AttributesFormatString=out（标定处理器温度输出（℃））
  wires:
  In1/1 -> Bit2V/1
  Sum of Elements1/1 -> out/1
  V25/1 -> Sum of Elements/2
  Sum of Elements/1 -> Divide/1
  " Avg_Slope"/1 -> Divide/2
  Divide/1 -> Sum of Elements1/1
  " Avg_Slope1"/1 -> Sum of Elements1/2
  Bit2V/1 -> Sum of Elements/1

== system turbo_controller/COMMRead_ISM/ISM/HuanSuanN ==
  note: 用总温修正原位转速
      |
      | 实际转速会随环境温度产生不同的工作含义。这里接收Origin_Nc_Filter的原位滤波转速N，以及Calib
      | rating_T0的摄氏总温T0，计算一个按参考温度归一化的转速。
      |
      | 先把摄氏温度变成绝对温度：Tk=273.15+T0，单位K。
      | 再计算温度比例的平方根，并乘实际转速：
      | 修正转速 = N × sqrt(288.15 / Tk)。
      | 最后Range把结果限制到0～75000。
      |
      | 例如T0=15 ℃时Tk=288.15 K，比例为1，修正前后相同；温度更低时比例大于1，温度更高时比例小于1
      | 。输入N与输出采用同一转速单位。
      |
      | 输出名为HuanSuanZhuanSu。当前它被SaveData和SendData取出，用于记录与回传，没有查到直接作为
      | 闭环反馈使用。闭环用的Nc_Filter是另一条滤波转速，不要把两者混成一个变量。
  In1 : Inport
      settings: AttributesFormatString=In1（物理转速输入（转每分））
  In2 : Inport  Port=2
      settings: AttributesFormatString=In2（入口总温输入（℃））
  Add : Sum
      settings: AttributesFormatString=Add（加法求和）
  Constant1 : Constant  Value=single(288.15)  OutDataTypeStr=single
      settings: AttributesFormatString=Constant1（标准参考总温288.15开尔文）
  Constant2 : Constant  Value=single(273.15)  OutDataTypeStr=single
      settings: AttributesFormatString=Constant2（摄氏转开尔文偏移273.15）
  Constant5 : Constant  Value=75000  OutDataTypeStr=single
      settings: AttributesFormatString=Constant5（修正转速上限75000）
  Constant6 : Constant  Value=0  OutDataTypeStr=single
      settings: AttributesFormatString=Constant6（修正转速下限零）
  Divide : Product  Inputs=*/
      settings: AttributesFormatString=Divide（除法）
  Product : Product
      settings: AttributesFormatString=Product（乘法）
  Range : Stateflow chart  Description=|  TreatAsAtomicUnit=on
      | 本实例把温度修正转速限制在0～75000 rpm。输出用于记录与回传；不是闭环PI所用的Nc_Filter。
      | 
      | 把一个数限制在允许范围内
      | 
      | 输入包括待处理值、允许下限和允许上限。先比较是否越过上限，越过就输出上限；未超过上限时再检查下限，小于下限就输出下限；落在范围内则原样通过。恰好等于边界的值也保留。
      | 
      | 计算式：输出 = min(max(输入，下限)，上限)。
      | 例如下限为0、上限为100时，输入120输出100，输入-5输出0，输入60输出60。这里不做平均、不计算变化速度，也不记住上一拍；它只防止当前数值越界。具体边界由父子系统连入，不能把此处的输出一律理解为百分比。
      settings: AttributesFormatString=Range（限幅或范围）
  Sqrt : Sqrt
      settings: AttributesFormatString=Sqrt（平方根）
  out : Outport
      settings: AttributesFormatString=out（温度修正转速输出）
  wires:
  Range/1(Out) -> out/1
  Constant5/1 -> Range/2(Max)
  Constant6/1 -> Range/3(Min)
  In1/1 -> Product/1
  Constant1/1 -> Divide/1
  In2/1 -> Add/2
  Constant2/1 -> Add/1
  Add/1 -> Divide/2
  Sqrt/1 -> Product/2
  Divide/1 -> Sqrt/1
  Product/1 -> Range/1(In)

== system turbo_controller/COMMRead_ISM/ISM/Origin_Nc_Filter ==
  note: 对原始转速做一阶低通，减小采样抖动
      |
      | 每次把本拍输入与上次滤波结果按比例相加：
      | 本拍输出=α×本拍输入+β×上次输出；
      | α=Ts/(T+Ts)，β=T/(T+Ts)。
      |
      | 当前T=0.067 s，Ts=Ts_ms/1000=0.02 s，因此α约0.229885、β约0.770115。新输入约占23%，旧结果
      | 约占77%。例如上次输出100、本次输入200，本次滤波结果约123，随后逐步靠近200。
      |
      | 它抑制快速波动，也会让真实变化稍有滞后；不负责把ADC计数变成物理量，也不单凭滤波判定传感器
      | 故障。输出送Origin_Nc_Filter，供控制及记录链路使用。
  In1 : Inport
      settings: AttributesFormatString=In1（输入1）
  Constant1 : Constant  Value=Ts_ms  OutDataTypeStr=single  SampleTime=-1
      settings: AttributesFormatString=Constant1（常量1）
  Constant2 : Constant  Value=1000  OutDataTypeStr=single  SampleTime=-1
      settings: AttributesFormatString=Constant2（常量2）
  Constant6 : Constant  Value=single(0.067)  OutDataTypeStr=single  SampleTime=-1
      settings: AttributesFormatString=Constant6（常量6）
  Divide : Product  Inputs=*/
      settings: AttributesFormatString=Divide（除法）
  Integer Delay1 : Delay  DelayLength=1  InitialCondition=0
      settings: AttributesFormatString=Integer Delay1（整数延迟1）
  Product2 : Product  RndMeth=Zero
      settings: AttributesFormatString=Product2（乘法2）
  Product3 : Product  RndMeth=Zero
      settings: AttributesFormatString=Product3（乘法3）
  Subsystem1 : Subsystem  Description=|
      | 计算低通滤波中新样本的权重
      | 
      | 输入T为滤波时间常数（s），T_Sampling为采样周期（s）。输出α=T_Sampling/(T+T_Sampling)，供父级乘以本拍的新输入。
      | 
      | 当前T=0.067、采样周期0.02，α=0.02/0.087≈0.229885。也就是每拍只采用约23%的新值，另外约77%由历史结果补足。时间常数越大，新值权重越小，结果越平稳但响应越慢。
      | 
      | 本模块只算一个无量纲系数，不含延迟，也不直接输出温度、压力或转速。两项时间输入必须使用同一单位。
      settings: AttributesFormatString=Subsystem1（子系统1）
      mask Display: disp('T_S\n---------------\nT_S + T')
  Subsystem2 : Subsystem  Description=|
      | 计算低通滤波中历史结果的权重
      | 
      | 输入T为时间常数，T_Sampling为采样周期，两者都用s。输出β=T/(T+T_Sampling)，供父级乘以上一次滤波结果。
      | 
      | 当前T=0.067、采样周期0.02，β≈0.770115；与另一支路新样本权重α≈0.229885相加为1。这样常值输入最终会稳定在原值，不会因为反复相加而不断放大。
      | 
      | 本模块只计算系数，历史结果由父级延迟块保存。若把20 ms误传成20 s，权重和滤波速度都会完全改变，因此父级先将Ts_ms除以1000。
      settings: AttributesFormatString=Subsystem2（子系统2）
      mask Display: disp('T\n---------------\nT_S + T')
  Sum3 : Sum  Inputs=|++
      settings: AttributesFormatString=Sum3（加法求和3）
  Out1 : Outport
      settings: AttributesFormatString=Out1（输出1）
  wires:
  Constant2/1 -> Divide/2
  Divide/1 -> Subsystem1/2(T_Sampling), Subsystem2/2(T_Sampling)  "T_S（采样周期）"
  Constant1/1 -> Divide/1
  Integer Delay1/1 -> Product3/1
  Subsystem2/1(Out) -> Product3/2
  Product3/1 -> Sum3/2
  Sum3/1 -> Out1/1, Integer Delay1/1
  Product2/1 -> Sum3/1
  Subsystem1/1(Out) -> Product2/2
  Constant6/1 -> Subsystem2/1(T), Subsystem1/1(T)  "T（滤波时间常数）"
  In1/1 -> Product2/1

== system turbo_controller/COMMRead_ISM/ISM/Subsystem2 ==
  note: 在滤波前检查排温是否超过930度
      |
      | 输入来自Calibrating_T4，是已经标定成℃、但还没有低通滤波的排温。Constant1给出930 ℃上限，X
      | lim_Xdot_Judge负责判断与恢复确认，Unit Delay1保存上一有效温度。
      |
      | 排温超过930 ℃时，图表置X_Flag_Locking，并把内部温度输出保持为上次有效值。恢复到上限内后不
      | 是立即清标志，而要经过连续确认，计数CNT_X大于5才解除。当前图表没有相邻温度变化率判断。
      |
      | 本层只把故障标志Flag_T4_ExtreFailure送出；图表的X_Out仅反馈到记忆块，没有替换AnalogFilter_
      | T4主温度路径。所以这不是“主排温被930限幅”的模块。
      |
      | 该标志进入Sensor总线，但当前没有查到下游Bus Selector取用。它具备检测计算，不能因此认定它已
      | 接上自动停车。
  In1 : Inport
      settings: AttributesFormatString=In1（输入1）
  Constant1 : Constant  Value=930  OutDataTypeStr=single  SampleTime=-1
      settings: AttributesFormatString=Constant1（常量1）
  Unit Delay1 : UnitDelay  SampleTime=-1  HasFrameUpgradeWarning=on
      settings: AttributesFormatString=Unit Delay1（单位延迟1）
  Xlim_Xdot_Judge : Stateflow chart  Description=|  RequirementInfo={} %GIDa_4108271f_7ba4_4664_8a98_d79c2ab86c3a  TreatAsAtomicUnit=on
      | 排温超限标志怎样置位和解除
      | 
      | 父级给本图三个量：本次排温X、上限X_ulim=930 ℃、上次接受的温度X_pre。本图有记忆，既判断当前值，也记住故障状态和恢复次数。
      | 
      | 当X超过上限时，置X_Flag_Locking=true，温度输出X_Out采用X_pre，并清恢复计数。这样一次异常不会覆盖内部保留的有效温度。
      | 当X重新回到允许上限内时，开始累计CNT_X；连续确认到CNT_X>5后，接受当前X并解除故障标志。确认未完成时沿图中的保持路径继续处理。
      | 
      | 这里的“5”是调用次数，不是5秒；本工程控制周期Ts_ms为20 ms。确切解除时刻还受先计数还是先比较的路径顺序影响。
      | 
      | 输出故障标志交给Sensor总线，温度输出仅供本图下一次保持。未使用的Xin_pre和突变计数已删除，因此不要把它解释成温度变化率故障检测。
      settings: AttributesFormatString=Xlim_Xdot_Judge（输入限值输入变化量判断）
  Flag_T4_ExtreFailure : Outport
      settings: AttributesFormatString=Flag_T4_ExtreFailure（标志排气温度极值故障）
  wires:
  In1/1 -> Xlim_Xdot_Judge/1(X)
  Constant1/1 -> Xlim_Xdot_Judge/2(X_ulim)
  Xlim_Xdot_Judge/2(X_Out) -> Unit Delay1/1
  Unit Delay1/1 -> Xlim_Xdot_Judge/3(X_pre)
  Xlim_Xdot_Judge/1(X_Flag_Locking) -> Flag_T4_ExtreFailure/1

== system turbo_controller/ESM/Flags/EngineClp ==
  note: 【本页库子系统中文说明】BiHuanZhiLing
      | 一、它做什么？
      | 这是“过不过这条线”的判断器。将输入与阈值 PG_Instr_CloseLoop 作 == 比较，关
      | 系成立输出真（1），否则输出假（0）。例如>=包含恰好等于，>则不包含。它只给出
      | 判断标志，不会自行限幅、报警、切换状态或操作阀门；后续逻辑决定如何使用。名称
      | 可能只是用途提示，实际判据以这里的关系和阈值为准。
      | 二、本实例当前参数
      | 比较关系：==
      | 比较阈值：PG_Instr_CloseLoop
      | 输出数据类型：布尔值，真或假
      | 零交叉检测：开启
      | 三、怎样继续学习？
      | 这是标准库子系统实例。中文说明放在使用它的父级页面，并同步存入本块Descriptio
      | n（模块说明）；官方库链接保留。先看本实例的输入来自哪里、输出交给谁，再结合
      | 以上参数理解作用。
  note: 产生进入闭环模式的允许条件
      |
      | 起动分支的阶段结果达到2时，产生Start到Clp条件；手动到Clp使用闭环命令判断；初始到Clp保留复
      | 位恢复有效条件。
      |
      | 同一个“进入闭环”请求，在不同来源模式下有不同条件，不能只看当前目标转速非零就进入闭环。本
      | 处只输出转换许可，StateTranslation还要结合当前状态决定采用哪条转换。当前恢复标志上层未启用
      | ，恢复进入闭环路径不会自动投入。
  note: BiHuanZhiLing
      | BiHuanZhiLing：只判断一个条件
      |
      | 把输入与3比较，使用关系“==”。成立输出1，不成立输出0；输出是判断标志，不是把输入缩放成该
      | 常数。
      |
      | 这里识别一种指令编码。判断成立只说明指令匹配；父级还会结合有效帧、当前模式或其他允许条件决
      | 定是否更新。实际驱动要继续经过控制与板级输出，不能把1理解为硬件执行回执。
  note: Compare
      | To Constant
      | CompareTo Constant：只判断一个条件
      |
      | 把输入与2比较，使用关系“==”。成立输出1，不成立输出0；输出是判断标志，不是把输入缩放成该
      | 常数。
      |
      | 比较门限用于父级的分支条件，没有滤波、延时确认或锁存。例如输入恰好等于门限时，“>=、<=、==
      | ”成立，“>、<”不成立。是否需要持续确认或同时满足其他条件，由父级连线决定。
  S_Flag_EnigneState : Inport
      settings: AttributesFormatString=S_Flag_EnigneState（发动机状态标志）
  S_Instr : Inport  Port=2
      settings: AttributesFormatString=S_Instr（指令）
  S_Flag_ECUReset : Inport  Port=3
      settings: AttributesFormatString=S_Flag_ECUReset（复位恢复标志）
  BiHuanZhiLing : simulink/Logic and Bit Operations/Compare To Constant  Description=|  relop===  const=PG_Instr_CloseLoop  OutDataTypeStr=boolean
      | BiHuanZhiLing：只判断一个条件
      | 
      | 把输入与3比较，使用关系“==”。成立输出1，不成立输出0；输出是判断标志，不是把输入缩放成该常数。
      | 
      | 这里识别一种指令编码。判断成立只说明指令匹配；父级还会结合有效帧、当前模式或其他允许条件决定是否更新。实际驱动要继续经过控制与板级输出，不能把1理解为硬件执行回执。
      settings: AttributesFormatString=BiHuanZhiLing（闭环指令）
  Compare To Constant : simulink/Logic and Bit Operations/Compare To Constant  Description=|  relop===  const=2  OutDataTypeStr=boolean
      | CompareTo Constant：只判断一个条件
      | 
      | 把输入与2比较，使用关系“==”。成立输出1，不成立输出0；输出是判断标志，不是把输入缩放成该常数。
      | 
      | 比较门限用于父级的分支条件，没有滤波、延时确认或锁存。例如输入恰好等于门限时，“>=、<=、==”成立，“>、<”不成立。是否需要持续确认或同时满足其他条件，由父级连线决定。
      settings: AttributesFormatString=Compare To Constant（比较到常量）
  Constant2 : Constant  Value=true  OutDataTypeStr=boolean  SampleTime=-1
      settings: AttributesFormatString=Constant2（常量2）
  Constant4 : Constant  Value=false  OutDataTypeStr=boolean  SampleTime=-1
      settings: AttributesFormatString=Constant4（常量4）
  Switch : Switch  Criteria=u2 ~= 0  SaturateOnIntegerOverflow=off  InputSameDT=off
      settings: AttributesFormatString=Switch（开关选择）
  S_Start2Clp : Outport
      settings: AttributesFormatString=S_Start2Clp（起动转闭环）
  S_Manual2Clp : Outport  Port=2
      settings: AttributesFormatString=S_Manual2Clp（手动转闭环）
  S_Origin2Clp : Outport  Port=3
      settings: AttributesFormatString=S_Origin2Clp（原位转闭环）
  wires:
  BiHuanZhiLing/1 -> S_Manual2Clp/1
  S_Instr/1 -> BiHuanZhiLing/1
  Compare To Constant/1 -> S_Start2Clp/1
  S_Flag_EnigneState/1 -> Compare To Constant/1
  Switch/1 -> S_Origin2Clp/1
  Constant4/1 -> Switch/3
  Constant2/1 -> Switch/1
  S_Flag_ECUReset/1 -> Switch/2

== system turbo_controller/ESM/Flags/EngineOrigin ==
  note: 判断停车结束后是否可以回到初始模式
      |
      | 只有StopFinish为真，且当前转速Nc≤20000 rpm，两项同时满足才输出Stop2Origin。停车图完成但转
      | 速仍很高时，不立即给出这个许可。
      |
      | 这里不主动制动，也不强迫传感器转速归零。“回初始”是控制流程退出停车模式，不等同于轴已经完
      | 全静止。StateTranslation在当前确实处于Stop时才会使用这条转换条件。
  S_Nc : Inport
      settings: AttributesFormatString=S_Nc（发动机反馈转速（转每分））
  S_StopFinish : Inport  Port=2
      settings: AttributesFormatString=S_StopFinish（停车完成）
  Constant4 : Constant  Value=20000  OutDataTypeStr=single  SampleTime=-1
      settings: AttributesFormatString=Constant4（常量4）
  Logical Operator1 : Logic  AllPortsSameDT=off  OutDataTypeStr=boolean
      settings: AttributesFormatString=Logical Operator1（逻辑运算1）
  Relational Operator1 : RelationalOperator  Operator=<=  OutDataTypeStr=boolean  InputSameDT=off
      settings: AttributesFormatString=Relational Operator1（关系比较运算1）
  S_Stop2Origin : Outport
      settings: AttributesFormatString=S_Stop2Origin（停车转原位）
  wires:
  S_Nc/1 -> Relational Operator1/1
  Constant4/1 -> Relational Operator1/2
  Relational Operator1/1 -> Logical Operator1/1
  Logical Operator1/1 -> S_Stop2Origin/1
  S_StopFinish/1 -> Logical Operator1/2

== system turbo_controller/ESM/Flags/EngineStart ==
  note: 【本页库子系统中文说明】QiDongZhiLing
      | 一、它做什么？
      | 这是“过不过这条线”的判断器。将输入与阈值 PG_Instr_Start 作 == 比较，关系成
      | 立输出真（1），否则输出假（0）。例如>=包含恰好等于，>则不包含。它只给出判断
      | 标志，不会自行限幅、报警、切换状态或操作阀门；后续逻辑决定如何使用。名称可能
      | 只是用途提示，实际判据以这里的关系和阈值为准。
      | 二、本实例当前参数
      | 比较关系：==
      | 比较阈值：PG_Instr_Start
      | 输出数据类型：布尔值，真或假
      | 零交叉检测：开启
      | 三、怎样继续学习？
      | 这是标准库子系统实例。中文说明放在使用它的父级页面，并同步存入本块Descriptio
      | n（模块说明）；官方库链接保留。先看本实例的输入来自哪里、输出交给谁，再结合
      | 以上参数理解作用。
  note: 判断能否开始普通起动
      |
      | 命令必须等于PG_Instr_Start，同时当前转速Nc≤13000 rpm。两项同时成立才输出Origin2Start；其
      | 他命令或转速过高时不允许这条转换。
      |
      | 这只是从初始模式进入普通起动的门槛。点火、建压、供油和退出电机由Start内部顺序图接着执行，
      | 不能把13000理解为起动完成转速。工程当前只保留普通Start，不含空气或丙烷起动分支。
  note: Compare
      | To Constant5
      | CompareTo Constant5：只判断一个条件
      |
      | 把输入与13000比较，使用关系“<=”。成立输出1，不成立输出0；输出是判断标志，不是把输入缩放
      | 成该常数。
      |
      | 比较门限用于父级的分支条件，没有滤波、延时确认或锁存。例如输入恰好等于门限时，“>=、<=、==
      | ”成立，“>、<”不成立。是否需要持续确认或同时满足其他条件，由父级连线决定。
  note: QiDongZhiLing
      | QiDongZhiLing：只判断一个条件
      |
      | 把输入与1比较，使用关系“==”。成立输出1，不成立输出0；输出是判断标志，不是把输入缩放成该
      | 常数。
      |
      | 这里识别一种指令编码。判断成立只说明指令匹配；父级还会结合有效帧、当前模式或其他允许条件决
      | 定是否更新。实际驱动要继续经过控制与板级输出，不能把1理解为硬件执行回执。
  S_Instr : Inport
      settings: AttributesFormatString=S_Instr（指令）
  S_Nc : Inport  Port=2
      settings: AttributesFormatString=S_Nc（发动机反馈转速（转每分））
  Compare To Constant5 : simulink/Logic and Bit Operations/Compare To Constant  Description=|  relop=<=  const=13000  OutDataTypeStr=boolean
      | CompareTo Constant5：只判断一个条件
      | 
      | 把输入与13000比较，使用关系“<=”。成立输出1，不成立输出0；输出是判断标志，不是把输入缩放成该常数。
      | 
      | 比较门限用于父级的分支条件，没有滤波、延时确认或锁存。例如输入恰好等于门限时，“>=、<=、==”成立，“>、<”不成立。是否需要持续确认或同时满足其他条件，由父级连线决定。
      settings: AttributesFormatString=Compare To Constant5（比较到常量5）
  Logical Operator2 : Logic  AllPortsSameDT=off  OutDataTypeStr=boolean
      settings: AttributesFormatString=Logical Operator2（逻辑运算2）
  QiDongZhiLing : simulink/Logic and Bit Operations/Compare To Constant  Description=|  relop===  const=PG_Instr_Start  OutDataTypeStr=boolean
      | QiDongZhiLing：只判断一个条件
      | 
      | 把输入与1比较，使用关系“==”。成立输出1，不成立输出0；输出是判断标志，不是把输入缩放成该常数。
      | 
      | 这里识别一种指令编码。判断成立只说明指令匹配；父级还会结合有效帧、当前模式或其他允许条件决定是否更新。实际驱动要继续经过控制与板级输出，不能把1理解为硬件执行回执。
      settings: AttributesFormatString=QiDongZhiLing（起动指令）
  S_Origin2Start : Outport
      settings: AttributesFormatString=S_Origin2Start（原位转起动）
  wires:
  S_Instr/1 -> QiDongZhiLing/1
  S_Nc/1 -> Compare To Constant5/1
  Logical Operator2/1 -> S_Origin2Start/1
  QiDongZhiLing/1 -> Logical Operator2/1
  Compare To Constant5/1 -> Logical Operator2/2
